simulink model "TrajectoryTracking_MPC"  (R2024b)
settings: Solver=ode4  StartTime=0.0  StopTime=T_end  FixedStep=Ts  RelTol=1e-3
InitFcn:
  | clear persistent_anim_update
values from neighbouring files (symbols this model uses):
  approach_dist = 0.08 * mapScale    [MPC_Setup.m]
  delta_max = deg2rad(30)    [MPC_Setup.m]
  ds_real = s_dense(2) - s_dense(1)    [MPC_Setup.m]
  Gamma = zeros(nx*N_p, nu*N_p)    [MPC_Setup.m]
  goal_tol = 1.0    (= 1)    [MPC_Setup.m]
  H_mpc = (H_mpc + H_mpc')/2    [MPC_Setup.m]
  L = 2.7    [MPC_Setup.m]    (also in mpc_viewer3d.m = D.lf + D.lr)
  lr = 1.35    [MPC_Setup.m]
  n_laps = 3    [MPC_Setup.m]
  N_p = 60    [MPC_Setup.m]
  Phi = zeros(nx*N_p, nx)    [MPC_Setup.m]
  Psi = zeros(nx*N_p, N_p)    [MPC_Setup.m]
  Qbar = kron(eye(N_p), Q)    [MPC_Setup.m]
  theta0 = theta_ref(idx0)    [MPC_Setup.m]
  Ts = 0.02    [MPC_Setup.m]    (also in mpc_viewer3d.m = (t(end) - t(1)) / (N - 1))
  v_const = 8    [MPC_Setup.m]
undefined symbols (not defined in the file or in its folder): A_in, ddelta_max, goal_x, goal_y, ref_kp, ref_th, ref_x, ref_y, x0_init, y0_init
settings Model: PacingRate=100  Creator=kasimesen  LastModifiedBy=kasimesen
settings DataIOCC: ReturnWorkspaceOutputs=off

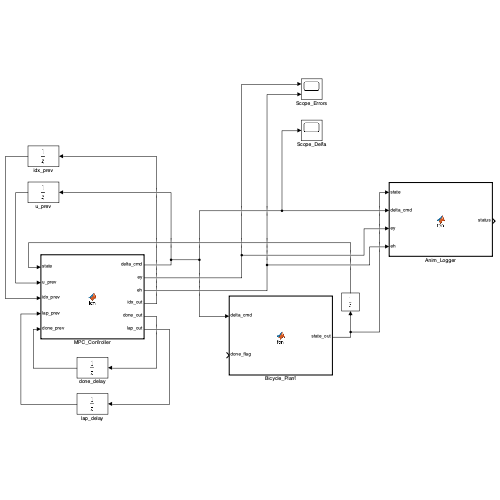
[thumbnail: Simulink's stored preview of the top-level diagram]
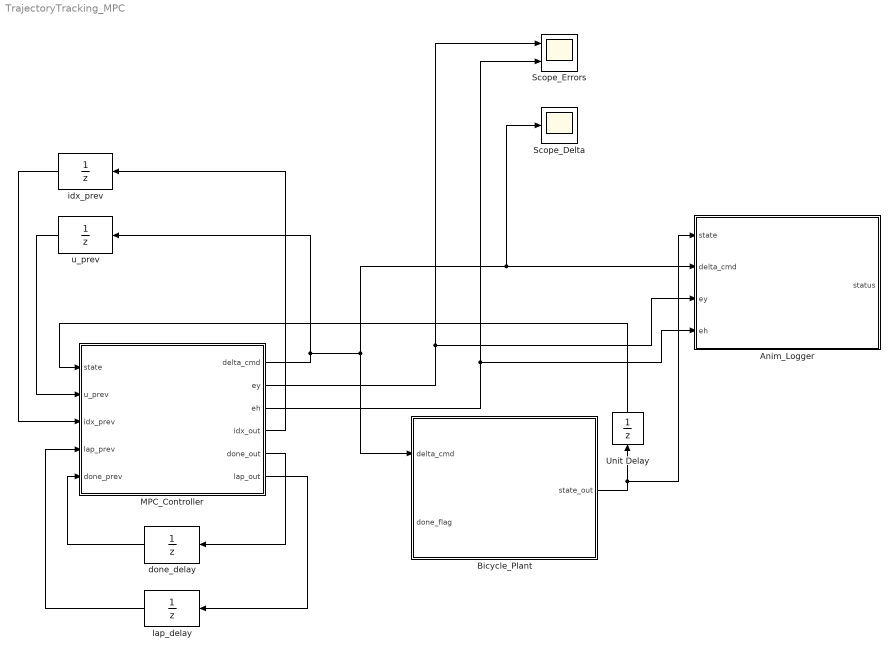
== system TrajectoryTracking_MPC ==
  Anim_Logger : MATLAB Function  TreatAsAtomicUnit=on
  Bicycle_Plant : MATLAB Function  TreatAsAtomicUnit=on
  MPC_Controller : MATLAB Function  TreatAsAtomicUnit=on
  Scope_Delta : Scope
  Scope_Errors : Scope  NumInputPorts=2
  Unit Delay : UnitDelay  SampleTime=Ts  HasFrameUpgradeWarning=on
  done_delay : UnitDelay  SampleTime=Ts  HasFrameUpgradeWarning=on
  idx_prev : UnitDelay  InitialCondition=1  SampleTime=Ts  HasFrameUpgradeWarning=on
  lap_delay : UnitDelay  SampleTime=Ts  HasFrameUpgradeWarning=on
  u_prev : UnitDelay  SampleTime=Ts  HasFrameUpgradeWarning=on
  wires:
  u_prev/1 -> MPC_Controller/2(u_prev)
  idx_prev/1 -> MPC_Controller/3(idx_prev)
  Bicycle_Plant/1(state_out) -> Unit Delay/1, Anim_Logger/1(state)
  MPC_Controller/1(delta_cmd) -> u_prev/1, Scope_Delta/1, Anim_Logger/2(delta_cmd), Bicycle_Plant/1(delta_cmd)
  MPC_Controller/2(ey) -> Scope_Errors/1, Anim_Logger/3(ey)
  MPC_Controller/3(eh) -> Scope_Errors/2, Anim_Logger/4(eh)
  MPC_Controller/4(idx_out) -> idx_prev/1
  Unit Delay/1 -> MPC_Controller/1(state)
  MPC_Controller/5(done_out) -> done_delay/1
  done_delay/1 -> MPC_Controller/5(done_prev)
  lap_delay/1 -> MPC_Controller/4(lap_prev)
  MPC_Controller/6(lap_out) -> lap_delay/1

== matlab function TrajectoryTracking_MPC/Bicycle_Plant ==
  data: delta_cmd input; state_out output; L parameter; lr parameter; v_const parameter; Ts parameter; x0_init parameter; y0_init parameter; theta0 parameter; done_flag input
function state_out = fcn(delta_cmd, L, lr, v_const, Ts, x0_init, y0_init, theta0, done_flag)
%#codegen
    persistent x y th initialized
    
    state_out = zeros(3,1);
    
    if isempty(initialized)
        x  = x0_init;
        y  = y0_init;
        th = theta0;
        initialized = true;
    end
    
    state_out = [x; y; th];
    

    if done_flag > 0.5
        return;
    end
    
    beta  = atan((lr/L)*tan(delta_cmd));
    xdot  = v_const*cos(th + beta);
    ydot  = v_const*sin(th + beta);
    thdot = (v_const/L)*cos(beta)*tan(delta_cmd);
    
    x  = x + xdot*Ts;
    y  = y + ydot*Ts;
    th = atan2(sin(th + thdot*Ts), cos(th + thdot*Ts));
end

== matlab function TrajectoryTracking_MPC/MPC_Controller ==
  data: state input; delta_cmd output; u_prev input; idx_prev input; ey output; eh output; idx_out output; ref_x parameter; ref_y parameter; ref_th parameter; ref_kp parameter; Phi parameter; Gamma parameter; Psi parameter; H_mpc parameter; A_in parameter; Qbar parameter; N_p parameter; v_const parameter; Ts parameter; delta_max parameter; ddelta_max parameter; approach_dist parameter; ds_real parameter; done_out output; goal_x parameter; goal_y parameter; goal_tol parameter; n_laps parameter; lap_prev input; done_prev input; lap_out output
function [delta_cmd, ey, eh, idx_out, done_out, lap_out] = fcn( ...
    state, u_prev, idx_prev, ref_x, ref_y, ref_th, ref_kp, ...
    Phi, Gamma, Psi, H_mpc, A_in, Qbar, ...
    N_p, v_const, Ts, delta_max, ddelta_max, approach_dist, ds_real, ...
    goal_x, goal_y, goal_tol, n_laps, lap_prev, done_prev) ...

    delta_cmd = double(u_prev);
    ey        = 0;
    eh        = 0;
    idx_out   = double(idx_prev);
    lap_out   = double(lap_prev);
    done_out  = double(done_prev);
    
    x  = state(1);
    y  = state(2);
    th = state(3);
    
    [delta_cmd, ey, eh, idx_out, lap_out, done_out] = mpc_solver( ...
        x, y, th, u_prev, ...
        ref_x, ref_y, ref_th, ref_kp, ...
        double(idx_prev), double(lap_prev), double(done_prev), ...
        Phi, Gamma, Psi, H_mpc, A_in, ...
        N_p, v_const, Ts, ...
        delta_max, ddelta_max, approach_dist, ...
        Qbar, ds_real, ...
        goal_x, goal_y, goal_tol, n_laps);
end

== matlab function TrajectoryTracking_MPC/Anim_Logger ==
  data: state input; status output; delta_cmd input; ey input; eh input
function status = fcn(state, delta_cmd, ey, eh)
    coder.extrinsic('persistent_anim_update');
    status = 0;
    persistent_anim_update(state(1), state(2), state(3), ...
                           delta_cmd, ey, eh);
end
